simulink model "demoDSRVdepthControl"  (R2022a)
settings: Solver=ode45  StartTime=0.0  StopTime=250  FixedStep=0.1  RelTol=1e-3  EnableMultiTasking=on
libraries: simulink_extras x2, mssSimulink x1, simulink x1
settings Model: Creator=thor  LastModifiedBy=thor
settings SolverCC: AlgebraicLoopSolver=TrustRegion
settings DataIOCC: LimitDataPoints=on  SaveFormat=Array  SignalLoggingSaveFormat=ModelDataLogs  ReturnWorkspaceOutputs=off  SignalLoggingName=sigsOut
settings OptimizationCC: BooleanDataType=off  InitFltsAndDblsToZero=on  LifeSpan=inf
settings DebuggingCC: SaveWithParameterizedLinksMsg=none  UnderspecifiedInitializationDetection=Classic  MergeDetectMultiDrivingBlocksExec=none  SignalResolutionControl=TryResolveAllWithWarning  MultiTaskDSMMsg=warning  MultiTaskCondExecSysMsg=none  FcnCallInpInsideContextMsg=warning  UnconnectedInputMsg=warning  UnconnectedOutputMsg=warning  UnconnectedLineMsg=warning  SFUnexpectedBacktrackingDiag=warning  SFNoUnconditionalDefaultTransitionDiag=warning  SFExecutionAtInitializationDiag=none  SFMachineParentedDataDiag=warning  ArithmeticOperatorsInVariantConditions=warning
settings HardwareCC: ProdBitPerPointer=32  ProdBitPerSizeT=32  ProdBitPerPtrDiffT=32  ProdLargestAtomicFloat=None  ProdIntDivRoundTo=Undefined  ProdEndianess=Unspecified  ProdWordSize=32  ProdHWDeviceType=32-bit Generic  TargetUnknown=on
settings ModelReferenceCC: PropagateSignalLabelsOutOfModel=off
settings RTWCC: DLArmComputeVersion=19.05
settings CodeAppCC: StateflowObjectComments=on
settings GRTTargetCC: TargetFcnLib=ansi_tfl_tmw.mat  TargetLangStandard=C89/C90 (ANSI)  ModelReferenceCompliant=off  CombineOutputUpdateFcns=off  MatFileLogging=off  GRTInterface=on
settings ConfigComp: CovMetricSettings=dw  CovSaveCumulativeToWorkspaceVar=on  CovSaveSingleToWorkspaceVar=on

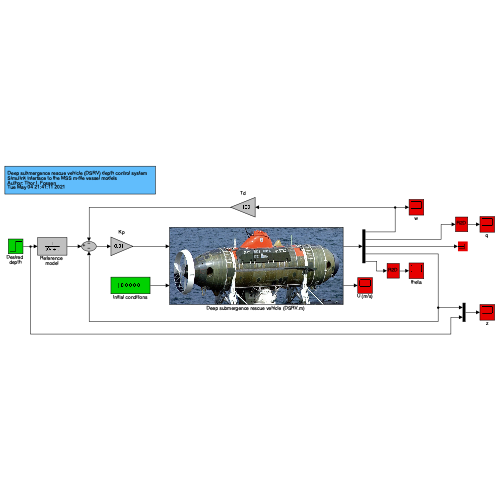
[thumbnail: Simulink's stored preview of the top-level diagram]
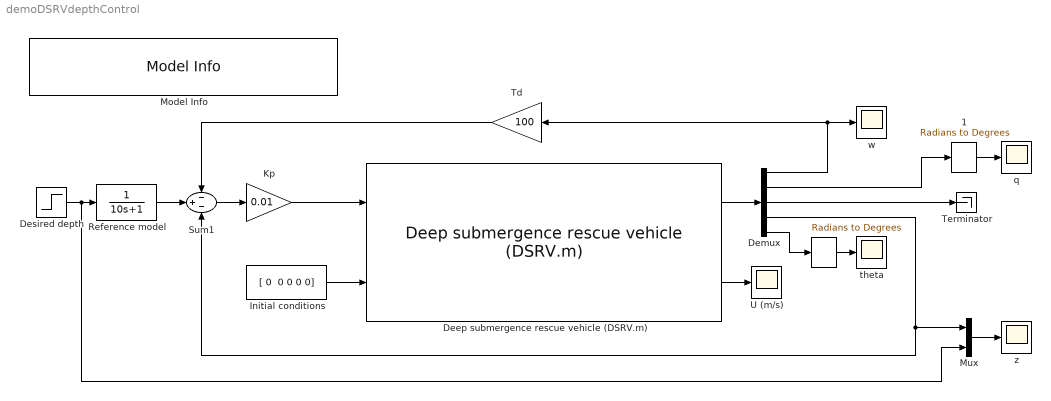
== system demoDSRVdepthControl ==
  "   " : simulink_extras/Transformations/Radians to Degrees
  "   1" : simulink_extras/Transformations/Radians to Degrees
  "Deep submergence rescue vehicle (DSRV.m) " : mssSimulink/Marine craft models/Deep submergence rescue vehicle (DSRV.m)  SystemSampleTime=-1  VariantActivationTime=update diagram  Latency=0  AutoFrameSizeCalculation=off
  Demux : Demux  Outputs=5
      settings: DisplayOption=none
  Desired depth : Step  Time=30  After=50  SampleTime=0
  Initial conditions : Constant  Value="[ 0  0 0 0 0]"
  Kp : Gain  Gain=0.01  SaturateOnIntegerOverflow=on  OutDataTypeStr=Inherit: Same as input  ParamDataTypeStr=Inherit: Same as input
  Model Info : simulink/Model-Wide Utilities/Model Info  Frame=on  DisplayStringWithTags=|  HorizontalTextAlignment=Left  LeftAlignmentValue=0.02
      | Deep submergence rescue vehicle (DSRV) depth control system
      | Simulink interface to the MSS m-file vessel models
      | Author: Thor I. Fossen
      | %<LastModificationDate>
  Mux : Mux  Inputs=2
  Reference model : TransferFcn  Denominator=[10 1]
  Sum1 : Sum  Inputs=-+-  InputSameDT=on  SaturateOnIntegerOverflow=on  OutDataTypeStr=Inherit: Same as first input
  Td : Gain  Gain=100  SaturateOnIntegerOverflow=on  OutDataTypeStr=Inherit: Same as input  ParamDataTypeStr=Inherit: Same as input
  Terminator : Terminator
  U (m/s) : Scope
  q : Scope
  theta : Scope
  w : Scope
  z : Scope
  wires:
  Initial conditions/1 -> "Deep submergence rescue vehicle (DSRV.m) "/2
  Demux/1 -> w/1, Td/1
  Demux/2 -> "   1"/1
  Kp/1 -> "Deep submergence rescue vehicle (DSRV.m) "/1
  Desired depth/1 -> Reference model/1, Mux/2
  Reference model/1 -> Sum1/2
  Sum1/1 -> Kp/1
  Td/1 -> Sum1/1
  "   "/1 -> theta/1
  "   1"/1 -> q/1
  Mux/1 -> z/1
  Demux/4 -> Mux/1, Sum1/3
  Demux/3 -> Terminator/1
  Demux/5 -> "   "/1
  "Deep submergence rescue vehicle (DSRV.m) "/1 -> Demux/1
  "Deep submergence rescue vehicle (DSRV.m) "/2 -> U (m/s)/1
